simulink model "freq_div"  (R2023a)
settings: Solver=VariableStepAuto  StartTime=0.0  StopTime=10.0  RelTol=1e-3
libraries: simulink x1
settings Model: Creator=mazen  LastModifiedBy=mazen

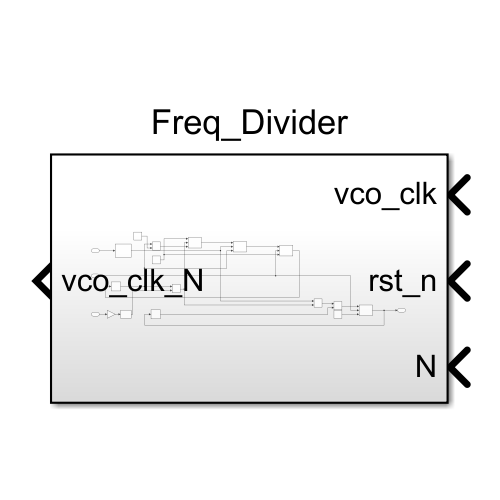
[thumbnail: Simulink's stored preview of the top-level diagram]
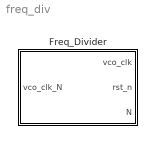
== system freq_div ==
  Freq_Divider : Subsystem

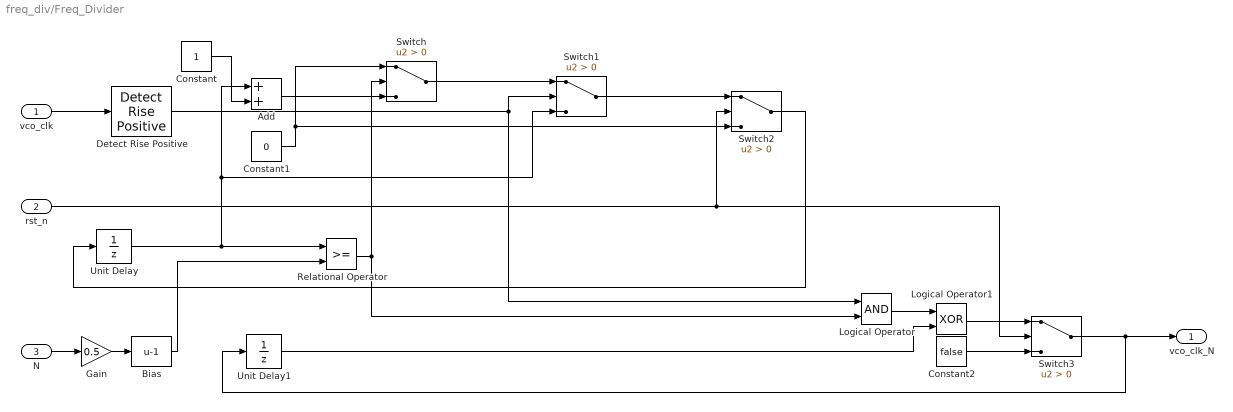
== system freq_div/Freq_Divider ==
  vco_clk : Inport
  rst_n : Inport  Port=2
  N : Inport  Port=3
  Add : Sum
  Bias : Bias  Bias=-1  SaturateOnIntegerOverflow=off
  Constant : Constant
  Constant1 : Constant  Value=0
  Constant2 : Constant  Value=false  OutDataTypeStr=boolean
  Detect Rise Positive : simulink/Logic and Bit Operations/Detect Rise Positive  vinit=0  OutDataTypeStr=boolean
  Gain : Gain  Gain=0.5
  Logical Operator : Logic  AllPortsSameDT=off  OutDataTypeStr=boolean
  Logical Operator1 : Logic  Operator=XOR  AllPortsSameDT=off  OutDataTypeStr=boolean
  Relational Operator : RelationalOperator  OutDataTypeStr=boolean  RndMeth=Simplest  InputSameDT=off
  Switch{,1..3} (4 alike) : Switch  Criteria=u2 > Threshold  SaturateOnIntegerOverflow=off  InputSameDT=off
  Unit Delay : UnitDelay  SampleTime=-1  HasFrameUpgradeWarning=on
  Unit Delay1 : UnitDelay  InitialCondition=false  SampleTime=-1  HasFrameUpgradeWarning=on
  vco_clk_N : Outport
  wires:
  Constant2/1 -> Switch3/3
  Switch2/1 -> Unit Delay/1
  Switch1/1 -> Switch2/1
  Add/1 -> Switch/3
  rst_n/1 -> Switch3/2, Switch2/2
  Relational Operator/1 -> Switch/2, Logical Operator/2
  Logical Operator/1 -> Logical Operator1/1
  Constant/1 -> Add/2
  Unit Delay/1 -> Relational Operator/1, Switch1/3, Add/1
  Constant1/1 -> Switch/1, Switch2/3
  vco_clk/1 -> Detect Rise Positive/1
  Gain/1 -> Bias/1
  Switch/1 -> Switch1/1
  Detect Rise Positive/1 -> Logical Operator/1, Switch1/2
  Logical Operator1/1 -> Switch3/1
  Switch3/1 -> Unit Delay1/1, vco_clk_N/1
  Unit Delay1/1 -> Logical Operator1/2
  Bias/1 -> Relational Operator/2
  N/1 -> Gain/1
